simulink model "robot_yorunge_denetimi"  (R2025b)
settings: Solver=ode4  StartTime=0.0  StopTime=3  FixedStep=0.01  RelTol=1e-3
settings Model: Creator=user  LastModifiedBy=user

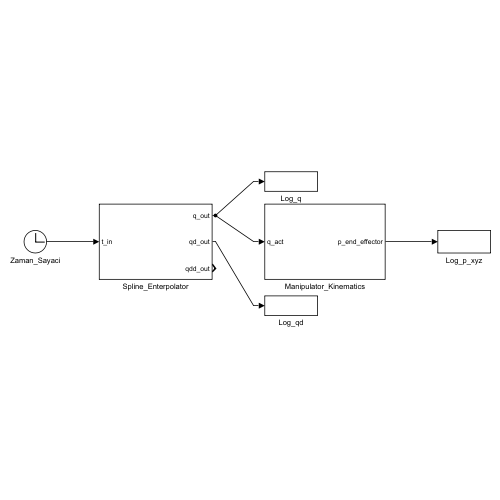
[thumbnail: Simulink's stored preview of the top-level diagram]
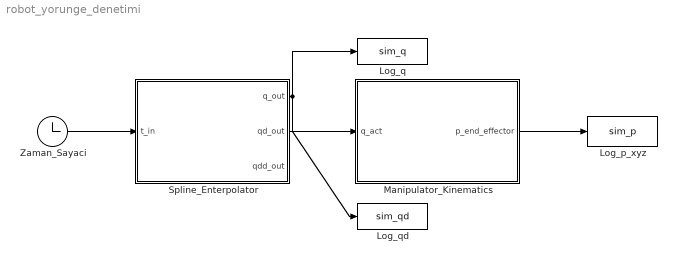
== system robot_yorunge_denetimi ==
  Log_p_xyz : ToWorkspace  VariableName=sim_p  SaveFormat=Timeseries  SampleTime=-1
  Log_q : ToWorkspace  VariableName=sim_q  SaveFormat=Timeseries  SampleTime=-1
  Log_qd : ToWorkspace  VariableName=sim_qd  SaveFormat=Timeseries  SampleTime=-1
  Manipulator_Kinematics : Subsystem
  Spline_Enterpolator : Subsystem
  Zaman_Sayaci : Clock
  wires:
  Zaman_Sayaci/1 -> Spline_Enterpolator/1(t_in)
  Spline_Enterpolator/1(q_out) -> Manipulator_Kinematics/1(q_act), Log_q/1
  Spline_Enterpolator/2(qd_out) -> Log_qd/1
  Manipulator_Kinematics/1(p_end_effector) -> Log_p_xyz/1

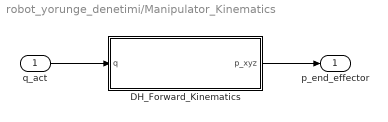
== system robot_yorunge_denetimi/Manipulator_Kinematics ==
  q_act : Inport
  DH_Forward_Kinematics : MATLAB Function  TreatAsAtomicUnit=on
  p_end_effector : Outport
  wires:
  q_act/1 -> DH_Forward_Kinematics/1(q)
  DH_Forward_Kinematics/1(p_xyz) -> p_end_effector/1

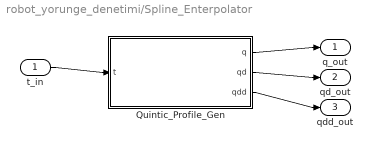
== system robot_yorunge_denetimi/Spline_Enterpolator ==
  t_in : Inport
  Quintic_Profile_Gen : MATLAB Function  TreatAsAtomicUnit=on
  q_out : Outport
  qd_out : Outport  Port=2
  qdd_out : Outport  Port=3
  wires:
  t_in/1 -> Quintic_Profile_Gen/1(t)
  Quintic_Profile_Gen/1(q) -> q_out/1
  Quintic_Profile_Gen/2(qd) -> qd_out/1
  Quintic_Profile_Gen/3(qdd) -> qdd_out/1

== matlab function robot_yorunge_denetimi/Spline_Enterpolator/Quintic_Profile_Gen ==
  data: t input; q output; qd output; qdd output
function [q, qd, qdd] = Quintic_Profile_Gen(t)
% 5. derece polinom enterpolasyonu
tf = 3.0000;
q0 = [0.000000; -0.785398; 1.047198; 0.000000; 0.523599; 0.000000];
qf = [1.047198; -0.523599; 0.785398; 0.785398; -0.785398; 1.570796];
tau = min(max(t / tf, 0), 1);
s   = 10*tau^3 - 15*tau^4 + 6*tau^5;
sd  = (30*tau^2 - 60*tau^3 + 30*tau^4) / tf;
sdd = (60*tau - 180*tau^2 + 120*tau^3) / (tf^2);
q   = q0 + (qf - q0) * s;
qd  = (qf - q0) * sd;
qdd = (qf - q0) * sdd;

== matlab function robot_yorunge_denetimi/Manipulator_Kinematics/DH_Forward_Kinematics ==
  data: q input; p_xyz output
function p_xyz = DH_Forward_Kinematics(q)
% DH parametreleri ile uç nokta kartezyen konumu hesabı
a = [0.0000, 0.4318, -0.0203, 0.0000, 0.0000, 0.0000];
alpha = [1.5708, 0.0000, -1.5708, 1.5708, -1.5708, 0.0000];
d = [0.6720, 0.0000, 0.1500, 0.4318, 0.0000, 0.0565];
T = eye(4);
for i = 1:6
    ct = cos(q(i)); st = sin(q(i)); ca = cos(alpha(i)); sa = sin(alpha(i));
    A = [ct, -st*ca,  st*sa, a(i)*ct;
         st,  ct*ca, -ct*sa, a(i)*st;
          0,     sa,     ca,    d(i);
          0,      0,      0,      1];
    T = T * A;
end
p_xyz = T(1:3, 4);
